simulink model "ieee33_bess_adaptive_R2022b"  (R2022b)
settings: Solver=ode3  StartTime=0  StopTime=4.5  FixedStep=5.0000000000000002e-05  RelTol=1e-3  EnableMultiTasking=on
libraries: spsThreePhaseSeriesRLCLoadLib x34, spsThreePhaseVIMeasurementLib x33, spsThreePhaseSeriesRLCBranchLib x32, spsThreePhaseDynamicLoadLib x2, spsRMSLib x2, spsGroundLib x1, spsPower3phInstantaneousLib x1, spsThreePhaseProgrammableVoltageSourceLib x1, spspowerguiLib x1
(part 2 of 2)

== matlab function ieee33_bess_adaptive_R2022b/Scenario Generator/Scenario Profile ==
  data: t input; Puv_W output; Quv_var output; Pover_W output; Qover_var output; scenarioId output; p input
function [Puv_W,Quv_var,Pover_W,Qover_var,scenarioId] = profile(t,p)
% p stores four [start end P18 Q18 P2 Q2] cases plus edge time.
Puv_W=0.0; Quv_var=0.0; Pover_W=0.0; Qover_var=0.0;
scenarioId=0.0; a=0.0; tr=max(p(25),1e-6);
if t>=p(1) && t<p(2)
    u=min(1.0,max(0.0,(t-p(1))/tr)); v=min(1.0,max(0.0,(p(2)-t)/tr));
    a=min(u*u*(3.0-2.0*u),v*v*(3.0-2.0*v));
    Puv_W=p(3)*a; Quv_var=p(4)*a; Pover_W=p(5)*a; Qover_var=p(6)*a; scenarioId=1.0;
elseif t>=p(7) && t<p(8)
    u=min(1.0,max(0.0,(t-p(7))/tr)); v=min(1.0,max(0.0,(p(8)-t)/tr));
    a=min(u*u*(3.0-2.0*u),v*v*(3.0-2.0*v));
    Puv_W=p(9)*a; Quv_var=p(10)*a; Pover_W=p(11)*a; Qover_var=p(12)*a; scenarioId=2.0;
elseif t>=p(13) && t<p(14)
    u=min(1.0,max(0.0,(t-p(13))/tr)); v=min(1.0,max(0.0,(p(14)-t)/tr));
    a=min(u*u*(3.0-2.0*u),v*v*(3.0-2.0*v));
    Puv_W=p(15)*a; Quv_var=p(16)*a; Pover_W=p(17)*a; Qover_var=p(18)*a; scenarioId=3.0;
elseif t>=p(19) && t<p(20)
    u=min(1.0,max(0.0,(t-p(19))/tr)); v=min(1.0,max(0.0,(p(20)-t)/tr));
    a=min(u*u*(3.0-2.0*u),v*v*(3.0-2.0*v));
    Puv_W=p(21)*a; Quv_var=p(22)*a; Pover_W=p(23)*a; Qover_var=p(24)*a; scenarioId=4.0;
end
end

== matlab function ieee33_bess_adaptive_R2022b/BESS Equivalent Model/BESS Step ==
  data: Pcmd input; stateNext output; Qcmd input; state input; Plim output; Qlim output; p input
function [stateNext,Plim,Qlim] = bess(Pcmd,Qcmd,state,p)
% p=[Ts Srated Pmax Qmax SOCmin SOCmax E etaDis etaCh tauP tauQ SbaseMW].
TS=p(1); SRATED=p(2); PMAX=p(3); QMAX=p(4); SOCMIN=p(5); SOCMAX=p(6);
E_MWH=p(7); ETA_DIS=p(8); ETA_CH=p(9); TAUP=max(p(10),TS); TAUQ=max(p(11),TS); SBASEMW=p(12);
Pess=state(1); Qess=state(2); SOC=state(3);
Qlim=min(QMAX,max(-QMAX,Qcmd));
Pavailable=min(PMAX,sqrt(max(SRATED*SRATED-Qlim*Qlim,0.0)));
Plim=min(Pavailable,max(-Pavailable,Pcmd));
if SOC<=SOCMIN && Plim>0.0; Plim=0.0; elseif SOC>=SOCMAX && Plim<0.0; Plim=0.0; end
aP=exp(-TS/TAUP); aQ=exp(-TS/TAUQ);
Pnext=aP*Pess+(1.0-aP)*Plim; Qnext=aQ*Qess+(1.0-aQ)*Qlim;
smag=sqrt(Pnext*Pnext+Qnext*Qnext);
if smag>SRATED; Pnext=Pnext/smag; Qnext=Qnext/smag; end
if SOC<=SOCMIN && Pnext>0.0; Pnext=0.0; elseif SOC>=SOCMAX && Pnext<0.0; Pnext=0.0; end
if Pnext>=0.0; dSOC=-(Pnext*SBASEMW/ETA_DIS)/(3600.0*E_MWH);
else; dSOC=-(ETA_CH*Pnext*SBASEMW)/(3600.0*E_MWH); end
SOCnext=min(SOCMAX,max(SOCMIN,SOC+TS*dSOC)); stateNext=[Pnext Qnext SOCnext];
end
